simulink model "cravoEcanela"  (R2024b)
settings: Solver=VariableStepAuto  StartTime=0.0  StopTime=simTim  RelTol=1e-3
values from neighbouring files (symbols this model uses):
  AGC_Target = -18    [romeuEjulieta.m]
  DRC_Threshold = -18    [romeuEjulieta.m]
  inputVolume = 1    [romeuEjulieta.m]
  noiseVolume = 0    [romeuEjulieta.m]
libraries: audiomeasurements x4, dspmathops x4, dspvision x2, commrfcorlib x1, audiodynamicrange x1, dspspect3 x1, dspsrcs4 x1
settings Model: Creator=Pedro  LastModifiedBy=Pedro

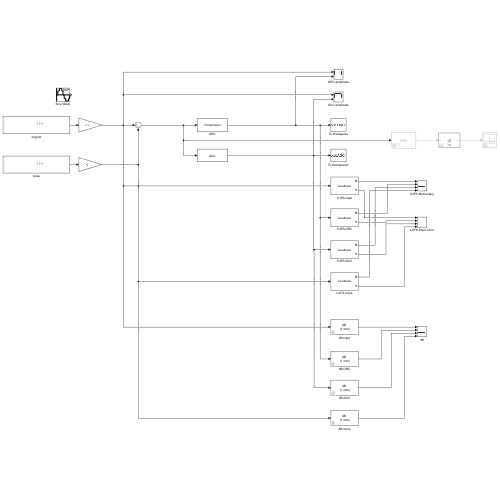
[thumbnail: Simulink's stored preview of the top-level diagram]
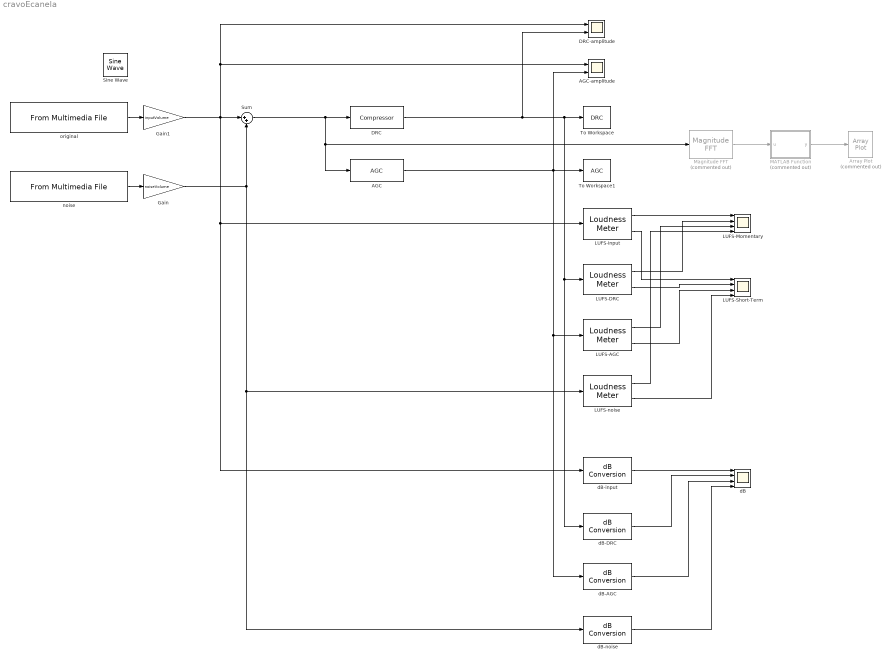
== system cravoEcanela ==
  AGC : commrfcorlib/AGC  LegacyMode=off  DetectorMethod=Rectifier  LoopMethod=Linear  UpdatePeriod=100  StepSize=0.1  AdaptationStepSize=AGC_Step_Size  DesiredOutputPower=10^(AGC_Target/10)  AveragingLength=AGC_Averging_Window_Length  MaximumGain=30  MaxPowerGain=AGC_Maximum_Power_Gain  GainOutputPort=off  InputPowerOutputPort=off  SimulateUsing=Code generation
  AGC-amplitude : Scope  NumInputPorts=2
  Array Plot : ArrayPlot  Commented=on  WindowPosition=[572.000000,160.000000,800.000000,687.000000,]  Visible=on  ScopeFrameLocation=window  SampleIncrement=10  AxesScaling=Manual  MaximizeAxes=Off  YLimits=[-15.7884 143.4193]
  DRC : audiodynamicrange/Compressor  ThresholdPort=off  Threshold=DRC_Threshold  RatioPort=off  Ratio=DRC_Ratio  KneeWidthPort=off  KneeWidth=DRC_Knee_Width  AttackTimePort=off  AttackTime=DRC_Attack_Time  ReleaseTimePort=off  ReleaseTime=DRC_Release_Time  MakeUpGainMode=Property  MakeUpGain=DRC_Make_up_Gain  InheritSampleRate=off  SampleRate=fs  outputGain=off  EnableSidechain=off  SimulateUsing=Interpreted execution
  DRC-amplitude : Scope  NumInputPorts=2
  Gain : Gain  Gain=noiseVolume
  Gain1 : Gain  Gain=inputVolume
  LUFS-AGC : audiomeasurements/Loudness Meter  ChannelWeights=[ 1, 1, 1, 1.41, 1.41 ]  UseRelativeScale=off  TargetLoudness=-23.0  OutputTruePeak=off  InheritSampleRate=off  SampleRate=fs  SimulateUsing=Interpreted execution
  LUFS-DRC : audiomeasurements/Loudness Meter  ChannelWeights=[ 1, 1, 1, 1.41, 1.41 ]  UseRelativeScale=off  TargetLoudness=-23.0  OutputTruePeak=off  InheritSampleRate=off  SampleRate=fs  SimulateUsing=Interpreted execution
  LUFS-Momentary : Scope  NumInputPorts=4
  LUFS-Short-Term : Scope  NumInputPorts=4
  LUFS-input : audiomeasurements/Loudness Meter  ChannelWeights=[ 1, 1, 1, 1.41, 1.41 ]  UseRelativeScale=off  TargetLoudness=-23.0  OutputTruePeak=off  InheritSampleRate=off  SampleRate=fs  SimulateUsing=Interpreted execution
  LUFS-noise : audiomeasurements/Loudness Meter  ChannelWeights=[ 1, 1, 1, 1.41, 1.41 ]  UseRelativeScale=off  TargetLoudness=-23.0  OutputTruePeak=off  InheritSampleRate=off  SampleRate=fs  SimulateUsing=Interpreted execution
  MATLAB Function : MATLAB Function  Commented=on  TreatAsAtomicUnit=on
  Magnitude FFT : dspspect3/Magnitude FFT  Commented=on  mag_or_magsq=Magnitude  FFTImplementation=Auto  fftLenInherit=off  fftsize=5000  WrapInput=off
  Sine Wave : dspsrcs4/Sine Wave  Amplitude=0.6  Frequency=100  Phase=0  SampleMode=Discrete  OutComplex=Real  CompMethod=Trigonometric fcn  TableSize=Speed  SampleTime=1/1000  SamplesPerFrame=1  ResetState=Restart at time zero  OutputFrames=off  dataType=double  wordLen=16  udDataType=sfix(16)  fracBitsMode=Best precision  numFracBits=15  OutDataTypeStr=double  LastOutDataTypeStr=double
  Sum : Sum  Inputs=|++
  To Workspace : ToWorkspace  VariableName=DRC  SampleTime=-1
      settings: Save2DSignal=2-D array (concatenate along first dimension)
  To Workspace1 : ToWorkspace  VariableName=AGC  SampleTime=-1
      settings: Save2DSignal=2-D array (concatenate along first dimension)
  dB : Scope  NumInputPorts=4
  dB-AGC : dspmathops/dB Conversion  dBtype=dB  intype=Amplitude  R=1  fuzz=off
      settings: LibrarySourceBlock=commutil2/dB Conversion
  dB-DRC : dspmathops/dB Conversion  dBtype=dB  intype=Amplitude  R=1  fuzz=off
      settings: LibrarySourceBlock=commutil2/dB Conversion
  dB-input : dspmathops/dB Conversion  dBtype=dB  intype=Amplitude  R=1  fuzz=off
      settings: LibrarySourceBlock=commutil2/dB Conversion
  dB-noise : dspmathops/dB Conversion  dBtype=dB  intype=Amplitude  R=1  fuzz=off
      settings: LibrarySourceBlock=commutil2/dB Conversion
  noise : dspvision/From Multimedia File  inputFilename=noise_track  readRange=[1 Inf]  loop=on  numPlays=inf  outputStreams=Audio only  videoDataType=single  audioDataType=double  inheritSampleTime=on  userDefinedSampleTime=1/30  noAudioOutput=off  isIntensityVideo=off  fourcc=RGB  colorVideoFormat=Separate color signals  outputEOF=off  dataOrg=Column-major  audioFrameSize=1024  computeAudioFrameSize=off  outSamplingMode=Sample based
      settings: LibrarySourceBlock=audiosources/From Multimedia File
  original : dspvision/From Multimedia File  inputFilename=input_track  readRange=[1 Inf]  loop=on  numPlays=1  outputStreams=Audio only  videoDataType=single  audioDataType=double  inheritSampleTime=on  userDefinedSampleTime=1/30  noAudioOutput=off  isIntensityVideo=off  fourcc=RGB  colorVideoFormat=Separate color signals  outputEOF=off  dataOrg=Column-major  audioFrameSize=1024  computeAudioFrameSize=off  outSamplingMode=Sample based
      settings: LibrarySourceBlock=audiosources/From Multimedia File
  wires:
  LUFS-input/1 -> LUFS-Momentary/1
  LUFS-DRC/1 -> LUFS-Momentary/2
  LUFS-AGC/1 -> LUFS-Momentary/3
  LUFS-input/2 -> LUFS-Short-Term/1
  LUFS-DRC/2 -> LUFS-Short-Term/2
  LUFS-AGC/2 -> LUFS-Short-Term/3
  dB-input/1 -> dB/1
  dB-DRC/1 -> dB/2
  dB-AGC/1 -> dB/3
  DRC/1 -> dB-DRC/1, LUFS-DRC/1, To Workspace/1, DRC-amplitude/2
  AGC/1 -> AGC-amplitude/2, dB-AGC/1, LUFS-AGC/1, To Workspace1/1
  Sum/1 -> Magnitude FFT/1, AGC/1, DRC/1
  Magnitude FFT/1 -> MATLAB Function/1(u)
  MATLAB Function/1(y) -> Array Plot/1
  original/1 -> Gain1/1
  noise/1 -> Gain/1
  Gain/1 -> dB-noise/1, LUFS-noise/1, Sum/2
  LUFS-noise/1 -> LUFS-Momentary/4
  LUFS-noise/2 -> LUFS-Short-Term/4
  dB-noise/1 -> dB/4
  Gain1/1 -> dB-input/1, LUFS-input/1, DRC-amplitude/1, AGC-amplitude/1, Sum/1

== matlab function cravoEcanela/MATLAB Function ==
  data: u input; y output
function y = fcn(u)

persistent buffer idx count;
N = 48000*0.1;

if isempty(buffer)
    buffer = zeros(N, 5000);
    idx = 1;
    count = 1;
end

buffer(idx,:) = u';
idx = idx + 1;

if idx > N
    idx = 1;
end

if count < N
    count = count + 1;
end

aux = sum(buffer,1)' ./ count;
y = aux(1:5000/2);
